simulink model "nms_sim_2D_cost"  (R2024b)
settings: Solver=ode15s  StartTime=0.0  StopTime=t_sim  MaxStep=dt_max  EnableMultiTasking=on
values from neighbouring files (symbols this model uses):
  a_BFSH = param_ctrl(35)*1    [setCtrlPar_optim_CPGreflex2001_2D.m]
  a_GAS = param_ctrl(37)*1    [setCtrlPar_optim_CPGreflex2001_2D.m]
  a_GLU = param_ctrl(31)*1    [setCtrlPar_optim_CPGreflex2001_2D.m]
  a_HAM = param_ctrl(33)*1    [setCtrlPar_optim_CPGreflex2001_2D.m]
  a_HFL = param_ctrl(32)*1    [setCtrlPar_optim_CPGreflex2001_2D.m]
  a_RF = param_ctrl(34)*1    [setCtrlPar_optim_CPGreflex2001_2D.m]
  a_SOL = param_ctrl(38)*1    [setCtrlPar_optim_CPGreflex2001_2D.m]
  a_TA = param_ctrl(39)*1    [setCtrlPar_optim_CPGreflex2001_2D.m]
  a_VAS = param_ctrl(36)*1    [setCtrlPar_optim_CPGreflex2001_2D.m]
  ai = param_ctrl(96)*2.0    [setCtrlPar_optim_CPGreflex2001_2D.m]
  b_BFSH = param_ctrl(52)*.51    [setCtrlPar_optim_CPGreflex2001_2D.m]
  b_BFSHGAS = param_ctrl(55)*.51    [setCtrlPar_optim_CPGreflex2001_2D.m]
  b_BFSHHAM = param_ctrl(54)*.51    [setCtrlPar_optim_CPGreflex2001_2D.m]
  b_BFSHVAS = param_ctrl(53)*.51    [setCtrlPar_optim_CPGreflex2001_2D.m]
  b_GAS = param_ctrl(59)*.51    [setCtrlPar_optim_CPGreflex2001_2D.m]
  b_GASBFSH = param_ctrl(60)*.51    [setCtrlPar_optim_CPGreflex2001_2D.m]
  b_GASSOL = param_ctrl(61)*.51    [setCtrlPar_optim_CPGreflex2001_2D.m]
  b_GLU = param_ctrl(40)*.51    [setCtrlPar_optim_CPGreflex2001_2D.m]
  b_GLUHAM = param_ctrl(42)*.51    [setCtrlPar_optim_CPGreflex2001_2D.m]
  b_GLUHFL = param_ctrl(41)*.51    [setCtrlPar_optim_CPGreflex2001_2D.m]
  b_HAM = param_ctrl(46)*.51    [setCtrlPar_optim_CPGreflex2001_2D.m]
  b_HAMBFSH = param_ctrl(48)*.51    [setCtrlPar_optim_CPGreflex2001_2D.m]
  b_HAMGLU = param_ctrl(47)*.51    [setCtrlPar_optim_CPGreflex2001_2D.m]
  b_HFL = param_ctrl(43)*.51    [setCtrlPar_optim_CPGreflex2001_2D.m]
  b_HFLGLU = param_ctrl(44)*.51    [setCtrlPar_optim_CPGreflex2001_2D.m]
  b_HFLRF = param_ctrl(45)*.51    [setCtrlPar_optim_CPGreflex2001_2D.m]
  b_RF = param_ctrl(49)*.51    [setCtrlPar_optim_CPGreflex2001_2D.m]
  b_RFHFL = param_ctrl(50)*.51    [setCtrlPar_optim_CPGreflex2001_2D.m]
  b_RFVAS = param_ctrl(51)*.51    [setCtrlPar_optim_CPGreflex2001_2D.m]
  b_SOL = param_ctrl(62)*.51    [setCtrlPar_optim_CPGreflex2001_2D.m]
  b_SOLGAS = param_ctrl(64)*.51    [setCtrlPar_optim_CPGreflex2001_2D.m]
  b_SOLTA = param_ctrl(63)*.51    [setCtrlPar_optim_CPGreflex2001_2D.m]
  b_TA = param_ctrl(65)*.51    [setCtrlPar_optim_CPGreflex2001_2D.m]
  b_TASOL = param_ctrl(66)*.51    [setCtrlPar_optim_CPGreflex2001_2D.m]
  b_VAS = param_ctrl(56)*.51    [setCtrlPar_optim_CPGreflex2001_2D.m]
  b_VASBFSH = param_ctrl(57)*.51    [setCtrlPar_optim_CPGreflex2001_2D.m]
  b_VASRF = param_ctrl(58)*.51    [setCtrlPar_optim_CPGreflex2001_2D.m]
  bias = param_ctrl(97)*2.5    [setCtrlPar_optim_CPGreflex2001_2D.m]
  c = 0.05    [nms_MS_2D_scaled.m]
  c_jointstop = 0.3 / (pi/180)    (= 17.1887338539)    [nms_MS_2D_scaled.m]
  D12_F = 0.16    *scaleL_JPhys    [nms_MechInit_2D_scaleSkel.m]
  D12_S = 0.2460	*sub_height    [nms_MechInit_2D_scaleSkel.m]
  D12_T = 0.2450  *sub_height    [nms_MechInit_2D_scaleSkel.m]
  D12y_F = 0.039  *sub_height    [nms_MechInit_2D_scaleSkel.m]
  D12z_HAT = 0.1    [nms_MS_2D_scaled.m]
  D13_F = 0.20    *scaleL_JPhys    [nms_MechInit_2D_scaleSkel.m]
  D1G_F = 0.14    *scaleL_JPhys    [nms_MechInit_2D_scaleSkel.m]
  D1G_HAT = 0.35  *scaleL_JPhys    [nms_MechInit_2D_scaleSkel.m]
  D1G_S = (0.3 - D12y_F/4)	*scaleL_JPhys    [nms_MechInit_2D_scaleSkel.m]
  D1G_T = (0.3 - D12y_F/4)	*scaleL_JPhys    [nms_MechInit_2D_scaleSkel.m]
  D1Gy_F = D12y_F*D1G_F/D12_F    (= 0.07)    [nms_MechInit_2D_scaleSkel.m]
  d_BFSH = param_ctrl(26)*1    [setCtrlPar_optim_CPGreflex2001_2D.m]
  d_GAS = param_ctrl(28)*1    [setCtrlPar_optim_CPGreflex2001_2D.m]
  d_GLU = param_ctrl(22)*1    [setCtrlPar_optim_CPGreflex2001_2D.m]
  d_HAM = param_ctrl(24)*1    [setCtrlPar_optim_CPGreflex2001_2D.m]
  d_HFL = param_ctrl(23)*1    [setCtrlPar_optim_CPGreflex2001_2D.m]
  d_RF = param_ctrl(25)*1    [setCtrlPar_optim_CPGreflex2001_2D.m]
  d_SOL = param_ctrl(29)*1    [setCtrlPar_optim_CPGreflex2001_2D.m]
  d_TA = param_ctrl(30)*1    [setCtrlPar_optim_CPGreflex2001_2D.m]
  d_VAS = param_ctrl(27)*1    [setCtrlPar_optim_CPGreflex2001_2D.m]
  DeltaThRef = 5e-3    (= 0.005)    [nms_MS_2D_scaled.m]
  dloptBFSH = 3.0    (= 3)    [setCtrlPar_optim_CPGreflex2001_2D.m]
  dloptGAS = 3.0    (= 3)    [setCtrlPar_optim_CPGreflex2001_2D.m]
  dloptGLU = 3.0    (= 3)    [setCtrlPar_optim_CPGreflex2001_2D.m]
  dloptHAM = 3.0    (= 3)    [setCtrlPar_optim_CPGreflex2001_2D.m]
  dloptHFL = 3.0    (= 3)    [setCtrlPar_optim_CPGreflex2001_2D.m]
  dloptRF = 3.0    (= 3)    [setCtrlPar_optim_CPGreflex2001_2D.m]
  dloptSOL = 3.0    (= 3)    [setCtrlPar_optim_CPGreflex2001_2D.m]
  dloptTA = 3.0    (= 3)    [setCtrlPar_optim_CPGreflex2001_2D.m]
  dloptVAS = 3.0    (= 3)    [setCtrlPar_optim_CPGreflex2001_2D.m]
  ec_BFSH = param_ctrl(80)*0.15    [setCtrlPar_optim_CPGreflex2001_2D.m]
  ec_GAS = param_ctrl(82)*0.15    [setCtrlPar_optim_CPGreflex2001_2D.m]
  ec_GLU = param_ctrl(76)*0.15    [setCtrlPar_optim_CPGreflex2001_2D.m]
  ec_HAM = param_ctrl(78)*0.15    [setCtrlPar_optim_CPGreflex2001_2D.m]
  ec_HFL = param_ctrl(77)*0.15    [setCtrlPar_optim_CPGreflex2001_2D.m]
  ec_RF = param_ctrl(79)*0.15    [setCtrlPar_optim_CPGreflex2001_2D.m]
  ec_TA = param_ctrl(84)*0.15    [setCtrlPar_optim_CPGreflex2001_2D.m]
  ec_VAS = param_ctrl(81)*0.15    [setCtrlPar_optim_CPGreflex2001_2D.m]
  eref = 0.04    [nms_MS_2D_scaled.m]
  eref_GAS = 0.1    [nms_MS_2D_scaled.m]
  eref_SOL = 0.1    [nms_MS_2D_scaled.m]
  es_BFSH = param_ctrl(89)*0.15    [setCtrlPar_optim_CPGreflex2001_2D.m]
  es_GAS = param_ctrl(91)*0.15    [setCtrlPar_optim_CPGreflex2001_2D.m]
  es_GLU = param_ctrl(85)*0.15    [setCtrlPar_optim_CPGreflex2001_2D.m]
  es_HAM = param_ctrl(87)*0.15    [setCtrlPar_optim_CPGreflex2001_2D.m]
  es_HFL = param_ctrl(86)*0.15    [setCtrlPar_optim_CPGreflex2001_2D.m]
  es_RF = param_ctrl(88)*0.15    [setCtrlPar_optim_CPGreflex2001_2D.m]
  es_TA = param_ctrl(93)*0.15    [setCtrlPar_optim_CPGreflex2001_2D.m]
  es_VAS = param_ctrl(90)*0.15    [setCtrlPar_optim_CPGreflex2001_2D.m]
  FmaxBFSH = 350    [nms_MS_2D_scaled.m]
  FmaxGAS = 2000    [nms_MS_2D_scaled.m]
  FmaxGLU = 4000    [nms_MS_2D_scaled.m]
  FmaxHAM = 2000    [nms_MS_2D_scaled.m]
  FmaxHFL = 2000    [nms_MS_2D_scaled.m]
  FmaxRF = 850    [nms_MS_2D_scaled.m]
  FmaxSOL = 4000    [nms_MS_2D_scaled.m]
  FmaxTA = 800    [nms_MS_2D_scaled.m]
  FmaxVAS = 5000    [nms_MS_2D_scaled.m]
  g = 9.81    [nms_MS_2D_scaled.m]
  gamma_4 = param_ctrl(11) * 1.7    [setCtrlPar_optim_CPGreflexsynergy2023_2D.m]
  h_BFSH = param_ctrl(71)*.1    [setCtrlPar_optim_CPGreflex2001_2D.m]
  h_GAS = param_ctrl(73)*.1    [setCtrlPar_optim_CPGreflex2001_2D.m]
  h_GLU = param_ctrl(67)*.1    [setCtrlPar_optim_CPGreflex2001_2D.m]
  h_HAM = param_ctrl(69)*.1    [setCtrlPar_optim_CPGreflex2001_2D.m]
  h_HFL = param_ctrl(68)*.1    [setCtrlPar_optim_CPGreflex2001_2D.m]
  h_RF = param_ctrl(70)*.1    [setCtrlPar_optim_CPGreflex2001_2D.m]
  h_SOL = param_ctrl(74)*.1    [setCtrlPar_optim_CPGreflex2001_2D.m]
  h_TA = param_ctrl(75)*.1    [setCtrlPar_optim_CPGreflex2001_2D.m]
  h_VAS = param_ctrl(72)*.1    [setCtrlPar_optim_CPGreflex2001_2D.m]
  HLCtrlPar = [theta_tgt l_clr alpha_tgt alpha_cd alpha_cv]    [setCtrlPar_optim_reflex2015_2D.m]
  In_F = 0.005    *scaleM*scaleL_JPhys^2    [nms_MechInit_2D_scaleSkel.m]
  In_HAT = 2.5    *scaleM*scaleL_JPhys^2    [nms_MechInit_2D_scaleSkel.m]
  In_S = 0.05     *scaleM*scaleL_JPhys^2    [nms_MechInit_2D_scaleSkel.m]
  In_T = 0.15     *scaleM*scaleL_JPhys^2    [nms_MechInit_2D_scaleSkel.m]
  init_exc = 0.01    [setInitPar_optim_2D.m]
  init_fm = 0.01    [setInitPar_optim_2D.m]
  init_lce = 1    [setInitPar_optim_2D.m]
  init_LCPG = param_ctrl(12) * 0.01    [setCtrlPar_optim_CPGreflexsynergy2023_2D.m]
  init_LStance = 1    [setInitPar_optim_2D.m]
  init_N1 = osc_signal1(phi_off_osc_ind)    [setCtrlPar_optim_CPGreflex2001_2D.m]
  ... (+441 more)
undefined symbols (not defined in the file or in its folder): cost_act_exponent, cost_v_tgt, flag_controller, Newton, nStep_obj, nStep_startKin, Raphson, sgn, SSW_kin, terrain_slope_angle, v_plateS1, X, Y, Z
libraries: nesl_utility x94, sm_lib x90, simulink x28, simulink_extras x12
(part 17 of 20)

== system nms_sim_2D_cost/Muscle Actuation/R SOL/CE force-length relation ==
  note: CE Force-Length Relationship
  lce [lopt] : Inport
  Abs : Abs  SaturateOnIntegerOverflow=off
  Constant1 : Constant
  Constant2 : Constant  Value=3
  Gain : Gain  Gain=log(c)
  Math Function : Math  SignedPower=on
  Math Function1 : Math  Operator=pow  SignedPower=on
  Sum4 : Sum  Inputs=|+-  InputSameDT=on  SaturateOnIntegerOverflow=on  OutDataTypeStr=Inherit: Same as first input
  normalized position : Product  Inputs=*/
  relative width : Constant  Value=w
  fce [Fmax] : Outport  VectorParamsAs1DForOutWhenUnconnected=off
  wires:
  lce [lopt]/1 -> Sum4/1
  relative width/1 -> normalized position/2
  Constant1/1 -> Sum4/2
  Sum4/1 -> Abs/1
  Abs/1 -> normalized position/1
  normalized position/1 -> Math Function1/1
  Constant2/1 -> Math Function1/2
  Math Function1/1 -> Gain/1
  Gain/1 -> Math Function/1
  Math Function/1 -> fce [Fmax]/1

== system nms_sim_2D_cost/Muscle Actuation/R SOL/CE inverse force-velocity relation ==
  note: CE Inverse Force-Velocity Relationship
  Fv[Fmax] : Inport
  1 : Product  Inputs=/*
  Constant{1,3..4,8} (4 alike) : Constant
  Constant2 : Constant  Value=N
  Constant5 : Constant  Value=N
  Curvature : Gain  Gain=K  SaturateOnIntegerOverflow=on  OutDataTypeStr=Inherit: Same as input  ParamDataTypeStr=Inherit: Same as input
  Curvature1 : Gain  Gain=7.56*K  SaturateOnIntegerOverflow=on  OutDataTypeStr=Inherit: Same as input  ParamDataTypeStr=Inherit: Same as input
  Mux : Mux  Inputs=2
  Mux1 : Mux  Inputs=3
  Mux2 : Mux  Inputs=3
  Slope : Gain  Gain=1e-2  SaturateOnIntegerOverflow=on  OutDataTypeStr=Inherit: Same as input  ParamDataTypeStr=Inherit: Same as input
  Sum1 : Sum  Inputs=|++  InputSameDT=on  SaturateOnIntegerOverflow=on  OutDataTypeStr=Inherit: Same as first input
  Sum2 : Sum  InputSameDT=on  SaturateOnIntegerOverflow=on  OutDataTypeStr=Inherit: Same as first input
  Sum3 : Sum  Inputs=++|  InputSameDT=on  SaturateOnIntegerOverflow=on  OutDataTypeStr=Inherit: Same as first input
  Sum4 : Sum  Inputs=|+-  InputSameDT=on  SaturateOnIntegerOverflow=on  OutDataTypeStr=Inherit: Same as first input
  Sum5 : Sum  Inputs=|-+  InputSameDT=on  SaturateOnIntegerOverflow=on  OutDataTypeStr=Inherit: Same as first input
  Sum6 : Sum  Inputs=-+|  InputSameDT=on  SaturateOnIntegerOverflow=on  OutDataTypeStr=Inherit: Same as first input
  Sum7 : Sum  Inputs=|++  InputSameDT=on  SaturateOnIntegerOverflow=on  OutDataTypeStr=Inherit: Same as first input
  Sum8 : Sum  Inputs=+-|  InputSameDT=on  SaturateOnIntegerOverflow=on  OutDataTypeStr=Inherit: Same as first input
  Sum9 : Sum  InputSameDT=on  SaturateOnIntegerOverflow=on  OutDataTypeStr=Inherit: Same as first input
  concentric branch : Fcn  Expr=u(1) * (u(2)<=1)
  excentric branch : Fcn  Expr=u(2) * (u(1)>1)*(u(1)<=u(3))
  excentric overshoot : Fcn  Expr=u(3) * (u(2)>u(1))
  v_concentric : Product  Inputs=*/
  v_excentric <N : Product  Inputs=*/
  v[vmax] : Outport  VectorParamsAs1DForOutWhenUnconnected=off
  wires:
  Curvature/1 -> Sum3/2
  Constant1/1 -> Sum4/2, Sum3/1
  Sum4/1 -> v_concentric/1
  Sum3/1 -> v_concentric/2
  1/1 -> Sum7/1, Curvature1/1
  Constant4/1 -> Sum7/2, Sum8/1
  Curvature1/1 -> Sum8/2
  Sum8/1 -> v_excentric <N/2
  Sum7/1 -> v_excentric <N/1
  v_concentric/1 -> Mux/1
  Fv[Fmax]/1 -> Sum4/1, Curvature/1, Sum6/2, Mux/2, Mux1/1, Mux2/2
  Sum9/1 -> v[vmax]/1
  Sum2/1 -> Sum9/2
  excentric overshoot/1 -> Sum2/2
  Slope/1 -> Sum1/1
  Constant8/1 -> Sum1/2
  Sum6/1 -> 1/2, Slope/1
  Constant2/1 -> Sum6/1, Sum5/2
  Sum5/1 -> 1/1
  Constant3/1 -> Sum5/1
  Mux/1 -> concentric branch/1
  Mux1/1 -> excentric branch/1
  v_excentric <N/1 -> Mux1/2
  Mux2/1 -> excentric overshoot/1
  concentric branch/1 -> Sum9/1
  excentric branch/1 -> Sum2/1
  Constant5/1 -> Mux1/3, Mux2/1
  Sum1/1 -> Mux2/3

== system nms_sim_2D_cost/Muscle Actuation/R SOL/PE force-length relation ==
  note: Parallel Elasticity PE
  lce [lopt] : Inport
  Constant3 : Constant
  Math Function2 : Math  Operator=square  SignedPower=on
  Mux : Mux  Inputs=2
  Sum1 : Sum  Inputs=|+-  InputSameDT=on  SaturateOnIntegerOverflow=on  OutDataTypeStr=Inherit: Same as first input
  force above slack length : Fcn  Expr=u(2) * (u(1)>1)
  reference strain [lopt] : Constant  Value=w_pe
  relative strain : Product  Inputs=*/
  fpe [Fmax] : Outport  VectorParamsAs1DForOutWhenUnconnected=off
  wires:
  Mux/1 -> force above slack length/1
  lce [lopt]/1 -> Mux/1, Sum1/1
  Constant3/1 -> Sum1/2
  Sum1/1 -> relative strain/1
  reference strain [lopt]/1 -> relative strain/2
  relative strain/1 -> Math Function2/1
  Math Function2/1 -> Mux/2
  force above slack length/1 -> fpe [Fmax]/1

== system nms_sim_2D_cost/Muscle Actuation/R SOL/SE force-length relation ==
  note: SE Force-Length Relationship
  lse [lslack] : Inport
  eref : Inport  Port=2
  Constant1 : Constant
  Math Function : Math  Operator=square  SignedPower=on
  Mux : Mux  Inputs=2
  Sum4 : Sum  Inputs=|+-  InputSameDT=on  SaturateOnIntegerOverflow=on  OutDataTypeStr=Inherit: Same as first input
  force above slack length : Fcn  Expr=u(2)*(u(1)>1)
  relative strain : Product  Inputs=*/
  fse [Fmax] : Outport  VectorParamsAs1DForOutWhenUnconnected=off
  wires:
  Mux/1 -> force above slack length/1
  force above slack length/1 -> fse [Fmax]/1
  Math Function/1 -> Mux/2
  lse [lslack]/1 -> Mux/1, Sum4/1
  relative strain/1 -> Math Function/1
  eref/1 -> relative strain/2
  Sum4/1 -> relative strain/1
  Constant1/1 -> Sum4/2

== system nms_sim_2D_cost/Muscle Actuation/RF/BE force-length relation ==
  note: Buffer Elasticity BE
  lce [lopt] : Inport
  Constant1 : Constant  Value=1-w
  Math Function : Math  Operator=square  SignedPower=on
  Mux1 : Mux  Inputs=2
  Sum4 : Sum  Inputs=|+-  InputSameDT=on  SaturateOnIntegerOverflow=on  OutDataTypeStr=Inherit: Same as first input
  force above slack length : Fcn  Expr=u(2)*(u(1)<0)
  reference strain [lslack] : Constant  Value=w/2
  relative strain : Product  Inputs=*/
  fbe [Fmax] : Outport  VectorParamsAs1DForOutWhenUnconnected=off
  wires:
  lce [lopt]/1 -> Sum4/1
  Mux1/1 -> force above slack length/1
  force above slack length/1 -> fbe [Fmax]/1
  Math Function/1 -> Mux1/2
  relative strain/1 -> Math Function/1
  reference strain [lslack]/1 -> relative strain/2
  Sum4/1 -> relative strain/1, Mux1/1
  Constant1/1 -> Sum4/2

== system nms_sim_2D_cost/Muscle Actuation/RF/CE force-length relation ==
  note: CE Force-Length Relationship
  lce [lopt] : Inport
  Abs : Abs  SaturateOnIntegerOverflow=off
  Constant1 : Constant
  Constant2 : Constant  Value=3
  Gain : Gain  Gain=log(c)
  Math Function : Math  SignedPower=on
  Math Function1 : Math  Operator=pow  SignedPower=on
  Sum4 : Sum  Inputs=|+-  InputSameDT=on  SaturateOnIntegerOverflow=on  OutDataTypeStr=Inherit: Same as first input
  normalized position : Product  Inputs=*/
  relative width : Constant  Value=w
  fce [Fmax] : Outport  VectorParamsAs1DForOutWhenUnconnected=off
  wires:
  lce [lopt]/1 -> Sum4/1
  relative width/1 -> normalized position/2
  Constant1/1 -> Sum4/2
  Sum4/1 -> Abs/1
  Abs/1 -> normalized position/1
  normalized position/1 -> Math Function1/1
  Constant2/1 -> Math Function1/2
  Math Function1/1 -> Gain/1
  Gain/1 -> Math Function/1
  Math Function/1 -> fce [Fmax]/1

== system nms_sim_2D_cost/Muscle Actuation/RF/CE inverse force-velocity relation ==
  note: CE Inverse Force-Velocity Relationship
  Fv[Fmax] : Inport
  1 : Product  Inputs=/*
  Constant{1,3..4,8} (4 alike) : Constant
  Constant2 : Constant  Value=N
  Constant5 : Constant  Value=N
  Curvature : Gain  Gain=K  SaturateOnIntegerOverflow=on  OutDataTypeStr=Inherit: Same as input  ParamDataTypeStr=Inherit: Same as input
  Curvature1 : Gain  Gain=7.56*K  SaturateOnIntegerOverflow=on  OutDataTypeStr=Inherit: Same as input  ParamDataTypeStr=Inherit: Same as input
  Mux : Mux  Inputs=2
  Mux1 : Mux  Inputs=3
  Mux2 : Mux  Inputs=3
  Slope : Gain  Gain=1e-2  SaturateOnIntegerOverflow=on  OutDataTypeStr=Inherit: Same as input  ParamDataTypeStr=Inherit: Same as input
  Sum1 : Sum  Inputs=|++  InputSameDT=on  SaturateOnIntegerOverflow=on  OutDataTypeStr=Inherit: Same as first input
  Sum2 : Sum  InputSameDT=on  SaturateOnIntegerOverflow=on  OutDataTypeStr=Inherit: Same as first input
  Sum3 : Sum  Inputs=++|  InputSameDT=on  SaturateOnIntegerOverflow=on  OutDataTypeStr=Inherit: Same as first input
  Sum4 : Sum  Inputs=|+-  InputSameDT=on  SaturateOnIntegerOverflow=on  OutDataTypeStr=Inherit: Same as first input
  Sum5 : Sum  Inputs=|-+  InputSameDT=on  SaturateOnIntegerOverflow=on  OutDataTypeStr=Inherit: Same as first input
  Sum6 : Sum  Inputs=-+|  InputSameDT=on  SaturateOnIntegerOverflow=on  OutDataTypeStr=Inherit: Same as first input
  Sum7 : Sum  Inputs=|++  InputSameDT=on  SaturateOnIntegerOverflow=on  OutDataTypeStr=Inherit: Same as first input
  Sum8 : Sum  Inputs=+-|  InputSameDT=on  SaturateOnIntegerOverflow=on  OutDataTypeStr=Inherit: Same as first input
  Sum9 : Sum  InputSameDT=on  SaturateOnIntegerOverflow=on  OutDataTypeStr=Inherit: Same as first input
  concentric branch : Fcn  Expr=u(1) * (u(2)<=1)
  excentric branch : Fcn  Expr=u(2) * (u(1)>1)*(u(1)<=u(3))
  excentric overshoot : Fcn  Expr=u(3) * (u(2)>u(1))
  v_concentric : Product  Inputs=*/
  v_excentric <N : Product  Inputs=*/
  v[vmax] : Outport  VectorParamsAs1DForOutWhenUnconnected=off
  wires:
  Curvature/1 -> Sum3/2
  Constant1/1 -> Sum4/2, Sum3/1
  Sum4/1 -> v_concentric/1
  Sum3/1 -> v_concentric/2
  1/1 -> Sum7/1, Curvature1/1
  Constant4/1 -> Sum7/2, Sum8/1
  Curvature1/1 -> Sum8/2
  Sum8/1 -> v_excentric <N/2
  Sum7/1 -> v_excentric <N/1
  v_concentric/1 -> Mux/1
  Fv[Fmax]/1 -> Sum4/1, Curvature/1, Sum6/2, Mux/2, Mux1/1, Mux2/2
  Sum9/1 -> v[vmax]/1
  Sum2/1 -> Sum9/2
  excentric overshoot/1 -> Sum2/2
  Slope/1 -> Sum1/1
  Constant8/1 -> Sum1/2
  Sum6/1 -> 1/2, Slope/1
  Constant2/1 -> Sum6/1, Sum5/2
  Sum5/1 -> 1/1
  Constant3/1 -> Sum5/1
  Mux/1 -> concentric branch/1
  Mux1/1 -> excentric branch/1
  v_excentric <N/1 -> Mux1/2
  Mux2/1 -> excentric overshoot/1
  concentric branch/1 -> Sum9/1
  excentric branch/1 -> Sum2/1
  Constant5/1 -> Mux1/3, Mux2/1
  Sum1/1 -> Mux2/3

== system nms_sim_2D_cost/Muscle Actuation/RF/PE force-length relation ==
  note: Parallel Elasticity PE
  lce [lopt] : Inport
  Constant3 : Constant
  Math Function2 : Math  Operator=square  SignedPower=on
  Mux : Mux  Inputs=2
  Sum1 : Sum  Inputs=|+-  InputSameDT=on  SaturateOnIntegerOverflow=on  OutDataTypeStr=Inherit: Same as first input
  force above slack length : Fcn  Expr=u(2) * (u(1)>1)
  reference strain [lopt] : Constant  Value=w_pe
  relative strain : Product  Inputs=*/
  fpe [Fmax] : Outport  VectorParamsAs1DForOutWhenUnconnected=off
  wires:
  Mux/1 -> force above slack length/1
  lce [lopt]/1 -> Mux/1, Sum1/1
  Constant3/1 -> Sum1/2
  Sum1/1 -> relative strain/1
  reference strain [lopt]/1 -> relative strain/2
  relative strain/1 -> Math Function2/1
  Math Function2/1 -> Mux/2
  force above slack length/1 -> fpe [Fmax]/1

== system nms_sim_2D_cost/Muscle Actuation/RF/SE force-length relation ==
  note: SE Force-Length Relationship
  lse [lslack] : Inport
  Constant1 : Constant
  Math Function : Math  Operator=square  SignedPower=on
  Mux : Mux  Inputs=2
  Sum4 : Sum  Inputs=|+-  InputSameDT=on  SaturateOnIntegerOverflow=on  OutDataTypeStr=Inherit: Same as first input
  force above slack length : Fcn  Expr=u(2)*(u(1)>1)
  reference strain [lslack] : Constant  Value=eref
  relative strain : Product  Inputs=*/
  fse [Fmax] : Outport  VectorParamsAs1DForOutWhenUnconnected=off
  wires:
  Mux/1 -> force above slack length/1
  force above slack length/1 -> fse [Fmax]/1
  Math Function/1 -> Mux/2
  lse [lslack]/1 -> Mux/1, Sum4/1
  relative strain/1 -> Math Function/1
  reference strain [lslack]/1 -> relative strain/2
  Sum4/1 -> relative strain/1
  Constant1/1 -> Sum4/2

== system nms_sim_2D_cost/Muscle Actuation/RF1/BE force-length relation ==
  note: Buffer Elasticity BE
  lce [lopt] : Inport
  Constant1 : Constant  Value=1-w
  Math Function : Math  Operator=square  SignedPower=on
  Mux1 : Mux  Inputs=2
  Sum4 : Sum  Inputs=|+-  InputSameDT=on  SaturateOnIntegerOverflow=on  OutDataTypeStr=Inherit: Same as first input
  force above slack length : Fcn  Expr=u(2)*(u(1)<0)
  reference strain [lslack] : Constant  Value=w/2
  relative strain : Product  Inputs=*/
  fbe [Fmax] : Outport  VectorParamsAs1DForOutWhenUnconnected=off
  wires:
  lce [lopt]/1 -> Sum4/1
  Mux1/1 -> force above slack length/1
  force above slack length/1 -> fbe [Fmax]/1
  Math Function/1 -> Mux1/2
  relative strain/1 -> Math Function/1
  reference strain [lslack]/1 -> relative strain/2
  Sum4/1 -> relative strain/1, Mux1/1
  Constant1/1 -> Sum4/2

== system nms_sim_2D_cost/Muscle Actuation/RF1/CE force-length relation ==
  note: CE Force-Length Relationship
  lce [lopt] : Inport
  Abs : Abs  SaturateOnIntegerOverflow=off
  Constant1 : Constant
  Constant2 : Constant  Value=3
  Gain : Gain  Gain=log(c)
  Math Function : Math  SignedPower=on
  Math Function1 : Math  Operator=pow  SignedPower=on
  Sum4 : Sum  Inputs=|+-  InputSameDT=on  SaturateOnIntegerOverflow=on  OutDataTypeStr=Inherit: Same as first input
  normalized position : Product  Inputs=*/
  relative width : Constant  Value=w
  fce [Fmax] : Outport  VectorParamsAs1DForOutWhenUnconnected=off
  wires:
  lce [lopt]/1 -> Sum4/1
  relative width/1 -> normalized position/2
  Constant1/1 -> Sum4/2
  Sum4/1 -> Abs/1
  Abs/1 -> normalized position/1
  normalized position/1 -> Math Function1/1
  Constant2/1 -> Math Function1/2
  Math Function1/1 -> Gain/1
  Gain/1 -> Math Function/1
  Math Function/1 -> fce [Fmax]/1

== system nms_sim_2D_cost/Muscle Actuation/RF1/CE inverse force-velocity relation ==
  note: CE Inverse Force-Velocity Relationship
  Fv[Fmax] : Inport
  1 : Product  Inputs=/*
  Constant{1,3..4,8} (4 alike) : Constant
  Constant2 : Constant  Value=N
  Constant5 : Constant  Value=N
  Curvature : Gain  Gain=K  SaturateOnIntegerOverflow=on  OutDataTypeStr=Inherit: Same as input  ParamDataTypeStr=Inherit: Same as input
  Curvature1 : Gain  Gain=7.56*K  SaturateOnIntegerOverflow=on  OutDataTypeStr=Inherit: Same as input  ParamDataTypeStr=Inherit: Same as input
  Mux : Mux  Inputs=2
  Mux1 : Mux  Inputs=3
  Mux2 : Mux  Inputs=3
  Slope : Gain  Gain=1e-2  SaturateOnIntegerOverflow=on  OutDataTypeStr=Inherit: Same as input  ParamDataTypeStr=Inherit: Same as input
  Sum1 : Sum  Inputs=|++  InputSameDT=on  SaturateOnIntegerOverflow=on  OutDataTypeStr=Inherit: Same as first input
  Sum2 : Sum  InputSameDT=on  SaturateOnIntegerOverflow=on  OutDataTypeStr=Inherit: Same as first input
  Sum3 : Sum  Inputs=++|  InputSameDT=on  SaturateOnIntegerOverflow=on  OutDataTypeStr=Inherit: Same as first input
  Sum4 : Sum  Inputs=|+-  InputSameDT=on  SaturateOnIntegerOverflow=on  OutDataTypeStr=Inherit: Same as first input
  Sum5 : Sum  Inputs=|-+  InputSameDT=on  SaturateOnIntegerOverflow=on  OutDataTypeStr=Inherit: Same as first input
  Sum6 : Sum  Inputs=-+|  InputSameDT=on  SaturateOnIntegerOverflow=on  OutDataTypeStr=Inherit: Same as first input
  Sum7 : Sum  Inputs=|++  InputSameDT=on  SaturateOnIntegerOverflow=on  OutDataTypeStr=Inherit: Same as first input
  Sum8 : Sum  Inputs=+-|  InputSameDT=on  SaturateOnIntegerOverflow=on  OutDataTypeStr=Inherit: Same as first input
  Sum9 : Sum  InputSameDT=on  SaturateOnIntegerOverflow=on  OutDataTypeStr=Inherit: Same as first input
  concentric branch : Fcn  Expr=u(1) * (u(2)<=1)
  excentric branch : Fcn  Expr=u(2) * (u(1)>1)*(u(1)<=u(3))
  excentric overshoot : Fcn  Expr=u(3) * (u(2)>u(1))
  v_concentric : Product  Inputs=*/
  v_excentric <N : Product  Inputs=*/
  v[vmax] : Outport  VectorParamsAs1DForOutWhenUnconnected=off
  wires:
  Curvature/1 -> Sum3/2
  Constant1/1 -> Sum4/2, Sum3/1
  Sum4/1 -> v_concentric/1
  Sum3/1 -> v_concentric/2
  1/1 -> Sum7/1, Curvature1/1
  Constant4/1 -> Sum7/2, Sum8/1
  Curvature1/1 -> Sum8/2
  Sum8/1 -> v_excentric <N/2
  Sum7/1 -> v_excentric <N/1
  v_concentric/1 -> Mux/1
  Fv[Fmax]/1 -> Sum4/1, Curvature/1, Sum6/2, Mux/2, Mux1/1, Mux2/2
  Sum9/1 -> v[vmax]/1
  Sum2/1 -> Sum9/2
  excentric overshoot/1 -> Sum2/2
  Slope/1 -> Sum1/1
  Constant8/1 -> Sum1/2
  Sum6/1 -> 1/2, Slope/1
  Constant2/1 -> Sum6/1, Sum5/2
  Sum5/1 -> 1/1
  Constant3/1 -> Sum5/1
  Mux/1 -> concentric branch/1
  Mux1/1 -> excentric branch/1
  v_excentric <N/1 -> Mux1/2
  Mux2/1 -> excentric overshoot/1
  concentric branch/1 -> Sum9/1
  excentric branch/1 -> Sum2/1
  Constant5/1 -> Mux1/3, Mux2/1
  Sum1/1 -> Mux2/3

== system nms_sim_2D_cost/Muscle Actuation/RF1/PE force-length relation ==
  note: Parallel Elasticity PE
  lce [lopt] : Inport
  Constant3 : Constant
  Math Function2 : Math  Operator=square  SignedPower=on
  Mux : Mux  Inputs=2
  Sum1 : Sum  Inputs=|+-  InputSameDT=on  SaturateOnIntegerOverflow=on  OutDataTypeStr=Inherit: Same as first input
  force above slack length : Fcn  Expr=u(2) * (u(1)>1)
  reference strain [lopt] : Constant  Value=w_pe
  relative strain : Product  Inputs=*/
  fpe [Fmax] : Outport  VectorParamsAs1DForOutWhenUnconnected=off
  wires:
  Mux/1 -> force above slack length/1
  lce [lopt]/1 -> Mux/1, Sum1/1
  Constant3/1 -> Sum1/2
  Sum1/1 -> relative strain/1
  reference strain [lopt]/1 -> relative strain/2
  relative strain/1 -> Math Function2/1
  Math Function2/1 -> Mux/2
  force above slack length/1 -> fpe [Fmax]/1

== system nms_sim_2D_cost/Muscle Actuation/RF1/SE force-length relation ==
  note: SE Force-Length Relationship
  lse [lslack] : Inport
  Constant1 : Constant
  Math Function : Math  Operator=square  SignedPower=on
  Mux : Mux  Inputs=2
  Sum4 : Sum  Inputs=|+-  InputSameDT=on  SaturateOnIntegerOverflow=on  OutDataTypeStr=Inherit: Same as first input
  force above slack length : Fcn  Expr=u(2)*(u(1)>1)
  reference strain [lslack] : Constant  Value=eref
  relative strain : Product  Inputs=*/
  fse [Fmax] : Outport  VectorParamsAs1DForOutWhenUnconnected=off
  wires:
  Mux/1 -> force above slack length/1
  force above slack length/1 -> fse [Fmax]/1
  Math Function/1 -> Mux/2
  lse [lslack]/1 -> Mux/1, Sum4/1
  relative strain/1 -> Math Function/1
  reference strain [lslack]/1 -> relative strain/2
  Sum4/1 -> relative strain/1
  Constant1/1 -> Sum4/2

== system nms_sim_2D_cost/Muscle Actuation/TA1/BE force-length relation ==
  note: Buffer Elasticity BE
  lce [lopt] : Inport
  Constant1 : Constant  Value=1-w
  Math Function : Math  Operator=square  SignedPower=on
  Mux1 : Mux  Inputs=2
  Sum4 : Sum  Inputs=|+-  InputSameDT=on  SaturateOnIntegerOverflow=on  OutDataTypeStr=Inherit: Same as first input
  force above slack length : Fcn  Expr=u(2)*(u(1)<0)
  reference strain [lslack] : Constant  Value=w/2
  relative strain : Product  Inputs=*/
  fbe [Fmax] : Outport  VectorParamsAs1DForOutWhenUnconnected=off
  wires:
  lce [lopt]/1 -> Sum4/1
  Mux1/1 -> force above slack length/1
  force above slack length/1 -> fbe [Fmax]/1
  Math Function/1 -> Mux1/2
  relative strain/1 -> Math Function/1
  reference strain [lslack]/1 -> relative strain/2
  Sum4/1 -> relative strain/1, Mux1/1
  Constant1/1 -> Sum4/2

== system nms_sim_2D_cost/Muscle Actuation/TA1/CE force-length relation ==
  note: CE Force-Length Relationship
  lce [lopt] : Inport
  Abs : Abs  SaturateOnIntegerOverflow=off
  Constant1 : Constant
  Constant2 : Constant  Value=3
  Gain : Gain  Gain=log(c)
  Math Function : Math  SignedPower=on
  Math Function1 : Math  Operator=pow  SignedPower=on
  Sum4 : Sum  Inputs=|+-  InputSameDT=on  SaturateOnIntegerOverflow=on  OutDataTypeStr=Inherit: Same as first input
  normalized position : Product  Inputs=*/
  relative width : Constant  Value=w
  fce [Fmax] : Outport  VectorParamsAs1DForOutWhenUnconnected=off
  wires:
  Math Function/1 -> fce [Fmax]/1
  Gain/1 -> Math Function/1
  Math Function1/1 -> Gain/1
  Constant2/1 -> Math Function1/2
  normalized position/1 -> Math Function1/1
  Abs/1 -> normalized position/1
  Sum4/1 -> Abs/1
  Constant1/1 -> Sum4/2
  relative width/1 -> normalized position/2
  lce [lopt]/1 -> Sum4/1

== system nms_sim_2D_cost/Muscle Actuation/TA1/CE inverse force-velocity relation ==
  note: CE Inverse Force-Velocity Relationship
  Fv[Fmax] : Inport
  1 : Product  Inputs=/*
  Constant{1,3..4,8} (4 alike) : Constant
  Constant2 : Constant  Value=N
  Constant5 : Constant  Value=N
  Curvature : Gain  Gain=K  SaturateOnIntegerOverflow=on  OutDataTypeStr=Inherit: Same as input  ParamDataTypeStr=Inherit: Same as input
  Curvature1 : Gain  Gain=7.56*K  SaturateOnIntegerOverflow=on  OutDataTypeStr=Inherit: Same as input  ParamDataTypeStr=Inherit: Same as input
  Mux : Mux  Inputs=2
  Mux1 : Mux  Inputs=3
  Mux2 : Mux  Inputs=3
  Slope : Gain  Gain=1e-2  SaturateOnIntegerOverflow=on  OutDataTypeStr=Inherit: Same as input  ParamDataTypeStr=Inherit: Same as input
  Sum1 : Sum  Inputs=|++  InputSameDT=on  SaturateOnIntegerOverflow=on  OutDataTypeStr=Inherit: Same as first input
  Sum2 : Sum  InputSameDT=on  SaturateOnIntegerOverflow=on  OutDataTypeStr=Inherit: Same as first input
  Sum3 : Sum  Inputs=++|  InputSameDT=on  SaturateOnIntegerOverflow=on  OutDataTypeStr=Inherit: Same as first input
  Sum4 : Sum  Inputs=|+-  InputSameDT=on  SaturateOnIntegerOverflow=on  OutDataTypeStr=Inherit: Same as first input
  Sum5 : Sum  Inputs=|-+  InputSameDT=on  SaturateOnIntegerOverflow=on  OutDataTypeStr=Inherit: Same as first input
  Sum6 : Sum  Inputs=-+|  InputSameDT=on  SaturateOnIntegerOverflow=on  OutDataTypeStr=Inherit: Same as first input
  Sum7 : Sum  Inputs=|++  InputSameDT=on  SaturateOnIntegerOverflow=on  OutDataTypeStr=Inherit: Same as first input
  Sum8 : Sum  Inputs=+-|  InputSameDT=on  SaturateOnIntegerOverflow=on  OutDataTypeStr=Inherit: Same as first input
  Sum9 : Sum  InputSameDT=on  SaturateOnIntegerOverflow=on  OutDataTypeStr=Inherit: Same as first input
  concentric branch : Fcn  Expr=u(1) * (u(2)<=1)
  excentric branch : Fcn  Expr=u(2) * (u(1)>1)*(u(1)<=u(3))
  excentric overshoot : Fcn  Expr=u(3) * (u(2)>u(1))
  v_concentric : Product  Inputs=*/
  v_excentric <N : Product  Inputs=*/
  v[vmax] : Outport  VectorParamsAs1DForOutWhenUnconnected=off
  wires:
  Sum1/1 -> Mux2/3
  Constant5/1 -> Mux2/1, Mux1/3
  excentric branch/1 -> Sum2/1
  concentric branch/1 -> Sum9/1
  Mux2/1 -> excentric overshoot/1
  v_excentric <N/1 -> Mux1/2
  Mux1/1 -> excentric branch/1
  Mux/1 -> concentric branch/1
  Constant3/1 -> Sum5/1
  Sum5/1 -> 1/1
  Constant2/1 -> Sum5/2, Sum6/1
  Sum6/1 -> Slope/1, 1/2
  Constant8/1 -> Sum1/2
  Slope/1 -> Sum1/1
  excentric overshoot/1 -> Sum2/2
  Sum2/1 -> Sum9/2
  Sum9/1 -> v[vmax]/1
  Fv[Fmax]/1 -> Mux2/2, Mux1/1, Mux/2, Sum6/2, Curvature/1, Sum4/1
  v_concentric/1 -> Mux/1
  Sum7/1 -> v_excentric <N/1
  Sum8/1 -> v_excentric <N/2
  Curvature1/1 -> Sum8/2
  Constant4/1 -> Sum8/1, Sum7/2
  1/1 -> Curvature1/1, Sum7/1
  Sum3/1 -> v_concentric/2
  Sum4/1 -> v_concentric/1
  Constant1/1 -> Sum3/1, Sum4/2
  Curvature/1 -> Sum3/2

== system nms_sim_2D_cost/Muscle Actuation/TA1/PE force-length relation ==
  note: Parallel Elasticity PE
  lce [lopt] : Inport
  Constant3 : Constant
  Math Function2 : Math  Operator=square  SignedPower=on
  Mux : Mux  Inputs=2
  Sum1 : Sum  Inputs=|+-  InputSameDT=on  SaturateOnIntegerOverflow=on  OutDataTypeStr=Inherit: Same as first input
  force above slack length : Fcn  Expr=u(2) * (u(1)>1)
  reference strain [lopt] : Constant  Value=w_pe
  relative strain : Product  Inputs=*/
  fpe [Fmax] : Outport  VectorParamsAs1DForOutWhenUnconnected=off
  wires:
  Mux/1 -> force above slack length/1
  lce [lopt]/1 -> Mux/1, Sum1/1
  Constant3/1 -> Sum1/2
  Sum1/1 -> relative strain/1
  reference strain [lopt]/1 -> relative strain/2
  relative strain/1 -> Math Function2/1
  Math Function2/1 -> Mux/2
  force above slack length/1 -> fpe [Fmax]/1

== system nms_sim_2D_cost/Muscle Actuation/TA1/SE force-length relation ==
  note: SE Force-Length Relationship
  lse [lslack] : Inport
  Constant1 : Constant
  Math Function : Math  Operator=square  SignedPower=on
  Mux : Mux  Inputs=2
  Sum4 : Sum  Inputs=|+-  InputSameDT=on  SaturateOnIntegerOverflow=on  OutDataTypeStr=Inherit: Same as first input
  force above slack length : Fcn  Expr=u(2)*(u(1)>1)
  reference strain [lslack] : Constant  Value=eref
  relative strain : Product  Inputs=*/
  fse [Fmax] : Outport  VectorParamsAs1DForOutWhenUnconnected=off
  wires:
  Mux/1 -> force above slack length/1
  force above slack length/1 -> fse [Fmax]/1
  Math Function/1 -> Mux/2
  lse [lslack]/1 -> Mux/1, Sum4/1
  relative strain/1 -> Math Function/1
  reference strain [lslack]/1 -> relative strain/2
  Sum4/1 -> relative strain/1
  Constant1/1 -> Sum4/2

== system nms_sim_2D_cost/Muscle Actuation/VAS/BE force-length relation ==
  note: Buffer Elasticity BE
  lce [lopt] : Inport
  Constant1 : Constant  Value=1-w
  Math Function : Math  Operator=square  SignedPower=on
  Mux1 : Mux  Inputs=2
  Sum4 : Sum  Inputs=|+-  InputSameDT=on  SaturateOnIntegerOverflow=on  OutDataTypeStr=Inherit: Same as first input
  force above slack length : Fcn  Expr=u(2)*(u(1)<0)
  reference strain [lslack] : Constant  Value=w/2
  relative strain : Product  Inputs=*/
  fbe [Fmax] : Outport  VectorParamsAs1DForOutWhenUnconnected=off
  wires:
  lce [lopt]/1 -> Sum4/1
  Mux1/1 -> force above slack length/1
  force above slack length/1 -> fbe [Fmax]/1
  Math Function/1 -> Mux1/2
  relative strain/1 -> Math Function/1
  reference strain [lslack]/1 -> relative strain/2
  Sum4/1 -> relative strain/1, Mux1/1
  Constant1/1 -> Sum4/2

== system nms_sim_2D_cost/Muscle Actuation/VAS/CE force-length relation ==
  note: CE Force-Length Relationship
  lce [lopt] : Inport
  Abs : Abs  SaturateOnIntegerOverflow=off
  Constant1 : Constant
  Constant2 : Constant  Value=3
  Gain : Gain  Gain=log(c)
  Math Function : Math  SignedPower=on
  Math Function1 : Math  Operator=pow  SignedPower=on
  Sum4 : Sum  Inputs=|+-  InputSameDT=on  SaturateOnIntegerOverflow=on  OutDataTypeStr=Inherit: Same as first input
  normalized position : Product  Inputs=*/
  relative width : Constant  Value=w
  fce [Fmax] : Outport  VectorParamsAs1DForOutWhenUnconnected=off
  wires:
  lce [lopt]/1 -> Sum4/1
  relative width/1 -> normalized position/2
  Constant1/1 -> Sum4/2
  Sum4/1 -> Abs/1
  Abs/1 -> normalized position/1
  normalized position/1 -> Math Function1/1
  Constant2/1 -> Math Function1/2
  Math Function1/1 -> Gain/1
  Gain/1 -> Math Function/1
  Math Function/1 -> fce [Fmax]/1

== system nms_sim_2D_cost/Muscle Actuation/VAS/CE inverse force-velocity relation ==
  note: CE Inverse Force-Velocity Relationship
  Fv[Fmax] : Inport
  1 : Product  Inputs=/*
  Constant{1,3..4,8} (4 alike) : Constant
  Constant2 : Constant  Value=N
  Constant5 : Constant  Value=N
  Curvature : Gain  Gain=K  SaturateOnIntegerOverflow=on  OutDataTypeStr=Inherit: Same as input  ParamDataTypeStr=Inherit: Same as input
  Curvature1 : Gain  Gain=7.56*K  SaturateOnIntegerOverflow=on  OutDataTypeStr=Inherit: Same as input  ParamDataTypeStr=Inherit: Same as input
  Mux : Mux  Inputs=2
  Mux1 : Mux  Inputs=3
  Mux2 : Mux  Inputs=3
  Slope : Gain  Gain=1e-2  SaturateOnIntegerOverflow=on  OutDataTypeStr=Inherit: Same as input  ParamDataTypeStr=Inherit: Same as input
  Sum1 : Sum  Inputs=|++  InputSameDT=on  SaturateOnIntegerOverflow=on  OutDataTypeStr=Inherit: Same as first input
  Sum2 : Sum  InputSameDT=on  SaturateOnIntegerOverflow=on  OutDataTypeStr=Inherit: Same as first input
  Sum3 : Sum  Inputs=++|  InputSameDT=on  SaturateOnIntegerOverflow=on  OutDataTypeStr=Inherit: Same as first input
  Sum4 : Sum  Inputs=|+-  InputSameDT=on  SaturateOnIntegerOverflow=on  OutDataTypeStr=Inherit: Same as first input
  Sum5 : Sum  Inputs=|-+  InputSameDT=on  SaturateOnIntegerOverflow=on  OutDataTypeStr=Inherit: Same as first input
  Sum6 : Sum  Inputs=-+|  InputSameDT=on  SaturateOnIntegerOverflow=on  OutDataTypeStr=Inherit: Same as first input
  Sum7 : Sum  Inputs=|++  InputSameDT=on  SaturateOnIntegerOverflow=on  OutDataTypeStr=Inherit: Same as first input
  Sum8 : Sum  Inputs=+-|  InputSameDT=on  SaturateOnIntegerOverflow=on  OutDataTypeStr=Inherit: Same as first input
  Sum9 : Sum  InputSameDT=on  SaturateOnIntegerOverflow=on  OutDataTypeStr=Inherit: Same as first input
  concentric branch : Fcn  Expr=u(1) * (u(2)<=1)
  excentric branch : Fcn  Expr=u(2) * (u(1)>1)*(u(1)<=u(3))
  excentric overshoot : Fcn  Expr=u(3) * (u(2)>u(1))
  v_concentric : Product  Inputs=*/
  v_excentric <N : Product  Inputs=*/
  v[vmax] : Outport  VectorParamsAs1DForOutWhenUnconnected=off
  wires:
  Curvature/1 -> Sum3/2
  Constant1/1 -> Sum4/2, Sum3/1
  Sum4/1 -> v_concentric/1
  Sum3/1 -> v_concentric/2
  1/1 -> Sum7/1, Curvature1/1
  Constant4/1 -> Sum7/2, Sum8/1
  Curvature1/1 -> Sum8/2
  Sum8/1 -> v_excentric <N/2
  Sum7/1 -> v_excentric <N/1
  v_concentric/1 -> Mux/1
  Fv[Fmax]/1 -> Sum4/1, Curvature/1, Sum6/2, Mux/2, Mux1/1, Mux2/2
  Sum9/1 -> v[vmax]/1
  Sum2/1 -> Sum9/2
  excentric overshoot/1 -> Sum2/2
  Slope/1 -> Sum1/1
  Constant8/1 -> Sum1/2
  Sum6/1 -> 1/2, Slope/1
  Constant2/1 -> Sum6/1, Sum5/2
  Sum5/1 -> 1/1
  Constant3/1 -> Sum5/1
  Mux/1 -> concentric branch/1
  Mux1/1 -> excentric branch/1
  v_excentric <N/1 -> Mux1/2
  Mux2/1 -> excentric overshoot/1
  concentric branch/1 -> Sum9/1
  excentric branch/1 -> Sum2/1
  Constant5/1 -> Mux1/3, Mux2/1
  Sum1/1 -> Mux2/3

== system nms_sim_2D_cost/Muscle Actuation/VAS/PE force-length relation ==
  note: Parallel Elasticity PE
  lce [lopt] : Inport
  Constant3 : Constant
  Math Function2 : Math  Operator=square  SignedPower=on
  Mux : Mux  Inputs=2
  Sum1 : Sum  Inputs=|+-  InputSameDT=on  SaturateOnIntegerOverflow=on  OutDataTypeStr=Inherit: Same as first input
  force above slack length : Fcn  Expr=u(2) * (u(1)>1)
  reference strain [lopt] : Constant  Value=w_pe
  relative strain : Product  Inputs=*/
  fpe [Fmax] : Outport  VectorParamsAs1DForOutWhenUnconnected=off
  wires:
  Mux/1 -> force above slack length/1
  lce [lopt]/1 -> Mux/1, Sum1/1
  Constant3/1 -> Sum1/2
  Sum1/1 -> relative strain/1
  reference strain [lopt]/1 -> relative strain/2
  relative strain/1 -> Math Function2/1
  Math Function2/1 -> Mux/2
  force above slack length/1 -> fpe [Fmax]/1

== system nms_sim_2D_cost/Muscle Actuation/VAS/SE force-length relation ==
  note: SE Force-Length Relationship
  lse [lslack] : Inport
  Constant1 : Constant
  Math Function : Math  Operator=square  SignedPower=on
  Mux : Mux  Inputs=2
  Sum4 : Sum  Inputs=|+-  InputSameDT=on  SaturateOnIntegerOverflow=on  OutDataTypeStr=Inherit: Same as first input
  force above slack length : Fcn  Expr=u(2)*(u(1)>1)
  reference strain [lslack] : Constant  Value=eref
  relative strain : Product  Inputs=*/
  fse [Fmax] : Outport  VectorParamsAs1DForOutWhenUnconnected=off
  wires:
  Mux/1 -> force above slack length/1
  force above slack length/1 -> fse [Fmax]/1
  Math Function/1 -> Mux/2
  lse [lslack]/1 -> Mux/1, Sum4/1
  relative strain/1 -> Math Function/1
  reference strain [lslack]/1 -> relative strain/2
  Sum4/1 -> relative strain/1
  Constant1/1 -> Sum4/2

== system nms_sim_2D_cost/Muscle Actuation/VAS1/BE force-length relation ==
  note: Buffer Elasticity BE
  lce [lopt] : Inport
  Constant1 : Constant  Value=1-w
  Math Function : Math  Operator=square  SignedPower=on
  Mux1 : Mux  Inputs=2
  Sum4 : Sum  Inputs=|+-  InputSameDT=on  SaturateOnIntegerOverflow=on  OutDataTypeStr=Inherit: Same as first input
  force above slack length : Fcn  Expr=u(2)*(u(1)<0)
  reference strain [lslack] : Constant  Value=w/2
  relative strain : Product  Inputs=*/
  fbe [Fmax] : Outport  VectorParamsAs1DForOutWhenUnconnected=off
  wires:
  lce [lopt]/1 -> Sum4/1
  Mux1/1 -> force above slack length/1
  force above slack length/1 -> fbe [Fmax]/1
  Math Function/1 -> Mux1/2
  relative strain/1 -> Math Function/1
  reference strain [lslack]/1 -> relative strain/2
  Sum4/1 -> relative strain/1, Mux1/1
  Constant1/1 -> Sum4/2

== system nms_sim_2D_cost/Muscle Actuation/VAS1/CE force-length relation ==
  note: CE Force-Length Relationship
  lce [lopt] : Inport
  Abs : Abs  SaturateOnIntegerOverflow=off
  Constant1 : Constant
  Constant2 : Constant  Value=3
  Gain : Gain  Gain=log(c)
  Math Function : Math  SignedPower=on
  Math Function1 : Math  Operator=pow  SignedPower=on
  Sum4 : Sum  Inputs=|+-  InputSameDT=on  SaturateOnIntegerOverflow=on  OutDataTypeStr=Inherit: Same as first input
  normalized position : Product  Inputs=*/
  relative width : Constant  Value=w
  fce [Fmax] : Outport  VectorParamsAs1DForOutWhenUnconnected=off
  wires:
  lce [lopt]/1 -> Sum4/1
  relative width/1 -> normalized position/2
  Constant1/1 -> Sum4/2
  Sum4/1 -> Abs/1
  Abs/1 -> normalized position/1
  normalized position/1 -> Math Function1/1
  Constant2/1 -> Math Function1/2
  Math Function1/1 -> Gain/1
  Gain/1 -> Math Function/1
  Math Function/1 -> fce [Fmax]/1

== system nms_sim_2D_cost/Muscle Actuation/VAS1/CE inverse force-velocity relation ==
  note: CE Inverse Force-Velocity Relationship
  Fv[Fmax] : Inport
  1 : Product  Inputs=/*
  Constant{1,3..4,8} (4 alike) : Constant
  Constant2 : Constant  Value=N
  Constant5 : Constant  Value=N
  Curvature : Gain  Gain=K  SaturateOnIntegerOverflow=on  OutDataTypeStr=Inherit: Same as input  ParamDataTypeStr=Inherit: Same as input
  Curvature1 : Gain  Gain=7.56*K  SaturateOnIntegerOverflow=on  OutDataTypeStr=Inherit: Same as input  ParamDataTypeStr=Inherit: Same as input
  Mux : Mux  Inputs=2
  Mux1 : Mux  Inputs=3
  Mux2 : Mux  Inputs=3
  Slope : Gain  Gain=1e-2  SaturateOnIntegerOverflow=on  OutDataTypeStr=Inherit: Same as input  ParamDataTypeStr=Inherit: Same as input
  Sum1 : Sum  Inputs=|++  InputSameDT=on  SaturateOnIntegerOverflow=on  OutDataTypeStr=Inherit: Same as first input
  Sum2 : Sum  InputSameDT=on  SaturateOnIntegerOverflow=on  OutDataTypeStr=Inherit: Same as first input
  Sum3 : Sum  Inputs=++|  InputSameDT=on  SaturateOnIntegerOverflow=on  OutDataTypeStr=Inherit: Same as first input
  Sum4 : Sum  Inputs=|+-  InputSameDT=on  SaturateOnIntegerOverflow=on  OutDataTypeStr=Inherit: Same as first input
  Sum5 : Sum  Inputs=|-+  InputSameDT=on  SaturateOnIntegerOverflow=on  OutDataTypeStr=Inherit: Same as first input
  Sum6 : Sum  Inputs=-+|  InputSameDT=on  SaturateOnIntegerOverflow=on  OutDataTypeStr=Inherit: Same as first input
  Sum7 : Sum  Inputs=|++  InputSameDT=on  SaturateOnIntegerOverflow=on  OutDataTypeStr=Inherit: Same as first input
  Sum8 : Sum  Inputs=+-|  InputSameDT=on  SaturateOnIntegerOverflow=on  OutDataTypeStr=Inherit: Same as first input
  Sum9 : Sum  InputSameDT=on  SaturateOnIntegerOverflow=on  OutDataTypeStr=Inherit: Same as first input
  concentric branch : Fcn  Expr=u(1) * (u(2)<=1)
  excentric branch : Fcn  Expr=u(2) * (u(1)>1)*(u(1)<=u(3))
  excentric overshoot : Fcn  Expr=u(3) * (u(2)>u(1))
  v_concentric : Product  Inputs=*/
  v_excentric <N : Product  Inputs=*/
  v[vmax] : Outport  VectorParamsAs1DForOutWhenUnconnected=off
  wires:
  Curvature/1 -> Sum3/2
  Constant1/1 -> Sum4/2, Sum3/1
  Sum4/1 -> v_concentric/1
  Sum3/1 -> v_concentric/2
  1/1 -> Sum7/1, Curvature1/1
  Constant4/1 -> Sum7/2, Sum8/1
  Curvature1/1 -> Sum8/2
  Sum8/1 -> v_excentric <N/2
  Sum7/1 -> v_excentric <N/1
  v_concentric/1 -> Mux/1
  Fv[Fmax]/1 -> Sum4/1, Curvature/1, Sum6/2, Mux/2, Mux1/1, Mux2/2
  Sum9/1 -> v[vmax]/1
  Sum2/1 -> Sum9/2
  excentric overshoot/1 -> Sum2/2
  Slope/1 -> Sum1/1
  Constant8/1 -> Sum1/2
  Sum6/1 -> 1/2, Slope/1
  Constant2/1 -> Sum6/1, Sum5/2
  Sum5/1 -> 1/1
  Constant3/1 -> Sum5/1
  Mux/1 -> concentric branch/1
  Mux1/1 -> excentric branch/1
  v_excentric <N/1 -> Mux1/2
  Mux2/1 -> excentric overshoot/1
  concentric branch/1 -> Sum9/1
  excentric branch/1 -> Sum2/1
  Constant5/1 -> Mux1/3, Mux2/1
  Sum1/1 -> Mux2/3

== system nms_sim_2D_cost/Muscle Actuation/VAS1/PE force-length relation ==
  note: Parallel Elasticity PE
  lce [lopt] : Inport
  Constant3 : Constant
  Math Function2 : Math  Operator=square  SignedPower=on
  Mux : Mux  Inputs=2
  Sum1 : Sum  Inputs=|+-  InputSameDT=on  SaturateOnIntegerOverflow=on  OutDataTypeStr=Inherit: Same as first input
  force above slack length : Fcn  Expr=u(2) * (u(1)>1)
  reference strain [lopt] : Constant  Value=w_pe
  relative strain : Product  Inputs=*/
  fpe [Fmax] : Outport  VectorParamsAs1DForOutWhenUnconnected=off
  wires:
  Mux/1 -> force above slack length/1
  lce [lopt]/1 -> Mux/1, Sum1/1
  Constant3/1 -> Sum1/2
  Sum1/1 -> relative strain/1
  reference strain [lopt]/1 -> relative strain/2
  relative strain/1 -> Math Function2/1
  Math Function2/1 -> Mux/2
  force above slack length/1 -> fpe [Fmax]/1

== system nms_sim_2D_cost/Muscle Actuation/VAS1/SE force-length relation ==
  note: SE Force-Length Relationship
  lse [lslack] : Inport
  Constant1 : Constant
  Math Function : Math  Operator=square  SignedPower=on
  Mux : Mux  Inputs=2
  Sum4 : Sum  Inputs=|+-  InputSameDT=on  SaturateOnIntegerOverflow=on  OutDataTypeStr=Inherit: Same as first input
  force above slack length : Fcn  Expr=u(2)*(u(1)>1)
  reference strain [lslack] : Constant  Value=eref
  relative strain : Product  Inputs=*/
  fse [Fmax] : Outport  VectorParamsAs1DForOutWhenUnconnected=off
  wires:
  Mux/1 -> force above slack length/1
  force above slack length/1 -> fse [Fmax]/1
  Math Function/1 -> Mux/2
  lse [lslack]/1 -> Mux/1, Sum4/1
  relative strain/1 -> Math Function/1
  reference strain [lslack]/1 -> relative strain/2
  Sum4/1 -> relative strain/1
  Constant1/1 -> Sum4/2

== system nms_sim_2D_cost/Muscle synergy Controller/Left Movement Regulator/Left Speed Regulator ==
  note: TA
  note: SOL
  v : Inport
  LStance1 : EnablePort
  Constant : Constant  Value=cost_v_tgt
  Constant1 : Constant  Value=lambda_TA
  Constant2 : Constant  Value=cost_v_tgt
  Constant3 : Constant  Value=lambda_SOL
  Gain : Gain  Gain=-1
  Gain1 : Gain  Gain=-1
  Product : Product
  Product1 : Product
  Sum : Sum  Inputs=|+-
  Sum1 : Sum  Inputs=|+-
  LExcTA_MR : Outport
  LExcSOL_MR : Outport  Port=2
  wires:
  Product/1 -> LExcTA_MR/1
  Gain/1 -> Product/2  "-lambda_TA"
  Sum/1 -> Product/1  "hip_speed - v_tgt"
  Constant/1 -> Sum/2
  Constant1/1 -> Gain/1
  v/1 -> Sum1/1, Sum/1
  Gain1/1 -> Product1/2  "-lambda_SOL"
  Sum1/1 -> Product1/1  "hip_speed - v_tgt"
  Product1/1 -> LExcSOL_MR/1
  Constant2/1 -> Sum1/2
  Constant3/1 -> Gain1/1

== system nms_sim_2D_cost/Muscle synergy Controller/Left Movement Regulator/Left Trunk Balance ==
  note: HFL
  note: GLU
  theta : Inport
  dtheta : Inport  Port=2
  LStance1 : EnablePort  StatesWhenEnabling=reset
  Constant : Constant  Value=theta_trunk_tgt
  Constant1 : Constant  Value=k_HFL
  Constant2 : Constant  Value=sigma_HFL
  Constant3 : Constant  Value=theta_trunk_tgt
  Constant4 : Constant  Value=k_GLU
  Constant5 : Constant  Value=sigma_GLU
  Gain : Gain  Gain=-1
  Gain1 : Gain  Gain=-1
  Product{,1..3} (4 alike) : Product
  Sum{,1..3} (4 alike) : Sum  Inputs=|+-
  LExcHFL_MR : Outport  OutputWhenDisabled=reset  InitialOutput=0
  LExcGLU_MR : Outport  Port=2
  wires:
  Sum1/1 -> LExcHFL_MR/1
  Constant1/1 -> Gain/1
  Constant2/1 -> Product1/1
  Gain/1 -> Product/2  "-K_HFL"
  Constant/1 -> Sum/2
  Product/1 -> Sum1/1
  Product1/1 -> Sum1/2
  Sum/1 -> Product/1  "theta - theta_tgt"
  Constant5/1 -> Product3/1
  Product2/1 -> Sum3/1
  Sum3/1 -> LExcGLU_MR/1
  Product3/1 -> Sum3/2
  Gain1/1 -> Product2/2  "-K_GLU"
  Sum2/1 -> Product2/1  "theta - theta_tgt"
  theta/1 -> Sum2/1, Sum/1
  Constant4/1 -> Gain1/1
  Constant3/1 -> Sum2/2
  dtheta/1 -> Product3/2, Product1/2

== system nms_sim_2D_cost/Muscle synergy Controller/Right Movement Regulator/Right Speed Regulator ==
  note: SOL
  note: TA
  v : Inport
  RStance : EnablePort
  Constant : Constant  Value=cost_v_tgt
  Constant1 : Constant  Value=lambda_TA
  Constant2 : Constant  Value=cost_v_tgt
  Constant3 : Constant  Value=lambda_SOL
  Gain : Gain  Gain=-1
  Gain1 : Gain  Gain=-1
  Product : Product
  Product1 : Product
  Sum : Sum  Inputs=|+-
  Sum1 : Sum  Inputs=|+-
  RExcTA_MR : Outport
  RExcSOL_MR : Outport  Port=2
  wires:
  Constant3/1 -> Gain1/1
  Constant2/1 -> Sum1/2
  Product1/1 -> RExcSOL_MR/1
  Sum1/1 -> Product1/1  "hip_speed - v_tgt"
  Gain1/1 -> Product1/2  "-lambda_SOL"
  v/1 -> Sum/1, Sum1/1
  Constant1/1 -> Gain/1
  Constant/1 -> Sum/2
  Sum/1 -> Product/1  "hip_speed - v_tgt"
  Gain/1 -> Product/2  "-lambda_TA"
  Product/1 -> RExcTA_MR/1
